simulink model "CLVF"  (R2020a)
settings: Solver=FixedStepAuto  StartTime=0.0  StopTime=tsim  FixedStep=baseRate  RelTol=1e-3  EnableMultiTasking=on
values from neighbouring files (symbols this model uses):
  a = sqrt(sum(aTimesOVec.^2))    [Run_Initializer.m]    (also in a_max_CLVF2D.m = params(4))
  a_max = 0.4/BLACKMass    [Run_Initializer.m]
  a_prime = newParams(2)    [Run_Initializer.m]    (also in a_max_LVF.m = params(2))
  acceptableRadius = 0.05    [Run_Initializer.m]
  b = newParams(3)    [Run_Initializer.m]    (also in a_max_CLVF2D.m = params(3))
  baseRate = 0.05    [Run_Initializer.m]
  BLACKMass = model_param(3)    [Run_Initializer.m]
  d = [0.16;0.542;0]    [Run_Initializer.m]    (also in a_max_LVF.m = [rotStuff(3);rotStuff(4);rotStuff(5)])
  drop_states_BLACK = rC_I0    [Run_Initializer.m]
  drop_states_BLUE = [ xLength/2+0.9; yLength/2+0.5; 0]    [Run_Initializer.m]
  drop_states_RED = rT_I0    [Run_Initializer.m]
  F_thrusters_BLACK = 0.25.*ones(8,1)    [Run_Initializer.m]
  F_thrusters_BLUE = 0.25.*ones(8,1)    [Run_Initializer.m]
  F_thrusters_RED = 0.25.*ones(8,1)    [Run_Initializer.m]
  home_states_BLACK = [ xLength/2+0.4; yLength/2; 0]    [Run_Initializer.m]
  home_states_BLUE = [ xLength/2-0.9; yLength/2+0.5; 0]    [Run_Initializer.m]
  home_states_RED = [ xLength/2-0.4; yLength/2; 0]    [Run_Initializer.m]
  init_states_BLACK = rC_I0    [Run_Initializer.m]
  init_states_BLUE = [ xLength/2+0.9; yLength/2+0.5; 0]    [Run_Initializer.m]
  init_states_RED = rT_I0    [Run_Initializer.m]
  k_v_rel = 2*v_max/a_prime    (= 1)    [Run_Initializer.m]
  ka = newParams(2)    [Run_Initializer.m]    (also in a_max_CLVF2D.m = params(2))
  kc = newParams(1)    [Run_Initializer.m]    (also in a_max_CLVF2D.m = params(1))
  kd = 5.0    (= 5)    [Run_Initializer.m]
  Kd_tb = 0.4    [Run_Initializer.m]
  Kd_tblue = 0.4    [Run_Initializer.m]
  Kd_tr = 0.4    [Run_Initializer.m]
  Kd_xb = 5    [Run_Initializer.m]
  Kd_xblue = 5    [Run_Initializer.m]
  Kd_xr = 5    [Run_Initializer.m]
  Kd_yb = 5    [Run_Initializer.m]
  Kd_yblue = 5    [Run_Initializer.m]
  Kd_yr = 5    [Run_Initializer.m]
  Kp_tb = 0.1    [Run_Initializer.m]
  Kp_tblue = 0.1    [Run_Initializer.m]
  Kp_tr = 0.1    [Run_Initializer.m]
  Kp_xb = 2    [Run_Initializer.m]
  Kp_xblue = 2    [Run_Initializer.m]
  Kp_xr = 2    [Run_Initializer.m]
  Kp_yb = 2    [Run_Initializer.m]
  Kp_yblue = 2    [Run_Initializer.m]
  Kp_yr = 2    [Run_Initializer.m]
  noise_variance_BLACK = 0    [Run_Initializer.m]
  noise_variance_BLUE = 0    [Run_Initializer.m]
  noise_variance_RED = 0    [Run_Initializer.m]
  o_hat_B = aTimesOVec./a    [Run_Initializer.m]
  o_hat_prime = o_prime/sqrt(sum(o_prime.^2))    [Run_Initializer.m]
  Phase0_End = Phase0_Duration    (= 10)    [Run_Initializer.m]
  Phase1_End = Phase0_Duration + Phase1_Duration    (= 15)    [Run_Initializer.m]
  Phase2_End = Phase0_Duration + Phase1_Duration +                                   Phase2_Duration    (= 35)    [Run_Initializer.m]
  Phase3_End = Phase0_Duration + Phase1_Duration +                                   Phase2_Duration + Phase3_Duration    [Run_Initializer.m]
  Phase3_SubPhase1_End = Phase2_End + Phase3_SubPhase1_Duration    (= 40)    [Run_Initializer.m]
  Phase3_SubPhase2_End = Phase2_End + Phase3_SubPhase1_Duration +                                   Phase3_SubPhase2_Duration    (= 45)    [Run_Initializer.m]
  Phase3_SubPhase3_End_BLACK = Phase2_End + Phase3_SubPhase1_Duration +                                   Phase3_SubPhase2_Duration +                                  Phase3_SubPhase3_Duration + Phase3_SubPhase3_and_a_half    (= 51)    [Run_Initializer.m]
  Phase3_SubPhase3_End_RED = Phase2_End + Phase3_SubPhase1_Duration +                                   Phase3_SubPhase2_Duration +                                  Phase3_SubPhase3_Duration    (= 46)    [Run_Initializer.m]
  Phase3_SubPhase4_End = Phase2_End + Phase3_SubPhase1_Duration +                                   Phase3_SubPhase2_Duration +                                  Phase3_SubPhase3_Duration +                                  Phase3_SubPhase4_Duration + Phase3_SubPhase3_and_a_half    [Run_Initializer.m]
  Phase4_End = Phase0_Duration + Phase1_Duration +                                   Phase2_Duration + Phase3_Duration +                                   Phase4_Duration    [Run_Initializer.m]
  Phase5_End = Phase0_Duration + Phase1_Duration +                                   Phase2_Duration + Phase3_Duration +                                   Phase4_Duration + Phase5_Duration    [Run_Initializer.m]
  r_co = r_co_over_a_prime*a_prime    (= 0.16)    [Run_Initializer.m]
  rC_I0 = [0.9*xLength;yLength/2-0.5;pi/2]    [Run_Initializer.m]
  rT_I0 = [yLength/2;yLength/2;possibleStarts(startingRotation)]    [Run_Initializer.m]
  serverRate = 0.1    [Run_Initializer.m]
  sys_BLACK = c2d(sys_BLACK_CONT, baseRate)    [Run_Initializer.m]
  sys_BLACK_ROT = c2d(sys_BLACK_rot_CONT, baseRate)    [Run_Initializer.m]
  sys_RED = c2d(sys_RED_CONT, baseRate)    [Run_Initializer.m]
  sys_RED_ROT = c2d(sys_RED_rot_CONT, baseRate)    [Run_Initializer.m]
  theta_d = 30*d2r    (= 0.523598775598)    [Run_Initializer.m]    (also in a_max_LVF.m = rotStuff(2))
  thruster_dist2CG_BLACK = [83.42;-52.58;55.94;-60.05;54.08;-53.92;77.06;-55.94]    [Run_Initializer.m]
  thruster_dist2CG_BLUE = [83.42;-52.58;55.94;-60.05;54.08;-53.92;77.06;-55.94]    [Run_Initializer.m]
  thruster_dist2CG_RED = [49.92;-78.08;70.46;-63.54;81.08;-50.42;57.44;-75.96]    [Run_Initializer.m]
  w_body = 6.0 * d2r    (= 0.10471975512)    [Run_Initializer.m]
undefined symbols (not defined in the file or in its folder): DiscIntNeverNeededParam, Discrete, Phase3_SubPhase3_End, platformSelection, simMode, Time, WhoAmI
libraries: dspstat3 x18, dspsigops x14, raspberrypiBasiclib x10, embdlinuxlib x8, simulink x8, ctrlSharedLib x4, mspfiltlib x3, dsparch4 x3, dspswit3 x2, MainLibrary x2, sensehatlib x1
(part 2 of 10)

== system CLVF/Phase #3: Experiment ==
  note: In this subsection, the "if" statements are used to determine two things: 1) whether or not a simulation is begin performed,
      | then 2) if an experiment is being performed, then which platform is the diagram compiled on. The "IdentifyPlatform" variable
      | is obtained from a text file location on each platform; each text file contains a unique identifier for each platform.
  Action Port : ActionPort  ActionPortLabel=elseif( u1 < u5)
  Change BLACK Behavior : Subsystem  TreatAsAtomicUnit=on
  Change BLUE Behavior : Subsystem  TreatAsAtomicUnit=on
  Change RED Behavior : Subsystem  TreatAsAtomicUnit=on
  Constant : Constant  Value=WhoAmI
  Is this a simulation? : Subsystem
  This IF block determines whether or not to run the BLACK sim/exp : If  NumInputs=2  IfExpression=u1 == 2 | u2 == 1  ShowElse=off
  This IF block determines whether or not to run the BLUE sim/exp : If  NumInputs=2  IfExpression=u1 == 3 | u2 == 1  ShowElse=off
  "This IF block determines whether or not to run the RED sim/exp " : If  NumInputs=2  IfExpression=u1 == 1 | u2 == 1  ShowElse=off
  wires:
  "This IF block determines whether or not to run the RED sim/exp "/1 -> Change RED Behavior/Action
  This IF block determines whether or not to run the BLACK sim/exp/1 -> Change BLACK Behavior/Action
  Constant/1 -> This IF block determines whether or not to run the BLUE sim/exp/1, This IF block determines whether or not to run the BLACK sim/exp/1, "This IF block determines whether or not to run the RED sim/exp "/1
  Is this a simulation?/1(isSim) -> This IF block determines whether or not to run the BLUE sim/exp/2, This IF block determines whether or not to run the BLACK sim/exp/2, "This IF block determines whether or not to run the RED sim/exp "/2
  This IF block determines whether or not to run the BLUE sim/exp/1 -> Change BLUE Behavior/Action

== system CLVF/Phase #4: Return Home ==
  note: In this subsection, the "if" statements are used to determine two things: 1) whether or not a simulation is begin performed,
      | then 2) if an experiment is being performed, then which platform is the diagram compiled on. The "IdentifyPlatform" variable
      | is obtained from a text file location on each platform; each text file contains a unique identifier for each platform.
  Action Port : ActionPort  ActionPortLabel=elseif( u1 < u6)
  Change BLACK Behavior : Subsystem  TreatAsAtomicUnit=on
  Change BLUE Behavior : Subsystem  TreatAsAtomicUnit=on
  Change RED Behavior : Subsystem  TreatAsAtomicUnit=on
  Constant : Constant  Value=WhoAmI
  Is this a simulation? : Subsystem
  This IF block determines whether or not to run the BLACK sim/exp : If  NumInputs=2  IfExpression=u1 == 2 | u2 == 1  ShowElse=off
  This IF block determines whether or not to run the BLUE sim/exp : If  NumInputs=2  IfExpression=u1 == 3 | u2 == 1  ShowElse=off
  "This IF block determines whether or not to run the RED sim/exp " : If  NumInputs=2  IfExpression=u1 == 1 | u2 == 1  ShowElse=off
  wires:
  "This IF block determines whether or not to run the RED sim/exp "/1 -> Change RED Behavior/Action
  This IF block determines whether or not to run the BLACK sim/exp/1 -> Change BLACK Behavior/Action
  Constant/1 -> This IF block determines whether or not to run the BLUE sim/exp/1, This IF block determines whether or not to run the BLACK sim/exp/1, "This IF block determines whether or not to run the RED sim/exp "/1
  Is this a simulation?/1(isSim) -> This IF block determines whether or not to run the BLUE sim/exp/2, This IF block determines whether or not to run the BLACK sim/exp/2, "This IF block determines whether or not to run the RED sim/exp "/2
  This IF block determines whether or not to run the BLUE sim/exp/1 -> Change BLUE Behavior/Action

== system CLVF/Phase #5: Hold Home ==
  note: In this subsection, the "if" statements are used to determine two things: 1) whether or not a simulation is begin performed,
      | then 2) if an experiment is being performed, then which platform is the diagram compiled on. The "IdentifyPlatform" variable
      | is obtained from a text file location on each platform; each text file contains a unique identifier for each platform.
  note: To change the behavior of RED during this phase, double click on the "Change RED Behavior". For BLACK, double click on "Change BLACK Behavior"
  Action Port : ActionPort  ActionPortLabel=elseif( u1 < u7 )
  Change BLACK Behavior : Subsystem  TreatAsAtomicUnit=on
  Change BLUE Behavior : Subsystem  TreatAsAtomicUnit=on
  Change RED Behavior : Subsystem  TreatAsAtomicUnit=on
  Constant : Constant  Value=WhoAmI
  Is this a simulation? : Subsystem
  This IF block determines whether or not to run the BLACK sim/exp : If  NumInputs=2  IfExpression=u1 == 2 | u2 == 1  ShowElse=off
  This IF block determines whether or not to run the BLUE sim/exp : If  NumInputs=2  IfExpression=u1 == 3 | u2 == 1  ShowElse=off
  "This IF block determines whether or not to run the RED sim/exp " : If  NumInputs=2  IfExpression=u1 == 1 | u2 == 1  ShowElse=off
  wires:
  "This IF block determines whether or not to run the RED sim/exp "/1 -> Change RED Behavior/Action
  This IF block determines whether or not to run the BLACK sim/exp/1 -> Change BLACK Behavior/Action
  Constant/1 -> This IF block determines whether or not to run the BLUE sim/exp/1, This IF block determines whether or not to run the BLACK sim/exp/1, "This IF block determines whether or not to run the RED sim/exp "/1
  This IF block determines whether or not to run the BLUE sim/exp/1 -> Change BLUE Behavior/Action
  Is this a simulation?/1(isSim) -> This IF block determines whether or not to run the BLACK sim/exp/2, This IF block determines whether or not to run the BLUE sim/exp/2, "This IF block determines whether or not to run the RED sim/exp "/2

== system CLVF/Phase #6: Stop Floating and Spin Down RW ==
  note: In this subsection, the "if" statements are used to determine two things: 1) whether or not a simulation is begin performed,
      | then 2) if an experiment is being performed, then which platform is the diagram compiled on. The "IdentifyPlatform" variable
      | is obtained from a text file location on each platform; each text file contains a unique identifier for each platform.
  Action Port : ActionPort  ActionPortLabel=else
  Change BLACK Behavior : Subsystem  TreatAsAtomicUnit=on
  Change BLUE Behavior : Subsystem  TreatAsAtomicUnit=on
  Change RED Behavior : Subsystem  TreatAsAtomicUnit=on
  Constant : Constant  Value=WhoAmI
  Is this a simulation? : Subsystem
  This IF block determines whether or not to run the BLACK sim/exp : If  NumInputs=2  IfExpression=u1 == 2 | u2 == 1  ShowElse=off
  This IF block determines whether or not to run the BLUE sim/exp : If  NumInputs=2  IfExpression=u1 == 3 | u2 == 1  ShowElse=off
  "This IF block determines whether or not to run the RED sim/exp " : If  NumInputs=2  IfExpression=u1 == 1 | u2 == 1  ShowElse=off
  wires:
  "This IF block determines whether or not to run the RED sim/exp "/1 -> Change RED Behavior/Action
  This IF block determines whether or not to run the BLACK sim/exp/1 -> Change BLACK Behavior/Action
  Is this a simulation?/1(isSim) -> This IF block determines whether or not to run the BLUE sim/exp/2, This IF block determines whether or not to run the BLACK sim/exp/2, "This IF block determines whether or not to run the RED sim/exp "/2
  This IF block determines whether or not to run the BLUE sim/exp/1 -> Change BLUE Behavior/Action
  Constant/1 -> This IF block determines whether or not to run the BLACK sim/exp/1, This IF block determines whether or not to run the BLUE sim/exp/1, "This IF block determines whether or not to run the RED sim/exp "/1

== system CLVF/Real-Time Visualization ==
  Set Universal Time (If this is a simulation) : Clock
  UDP Send : embdlinuxlib/UDP Send  remoteURL='192.168.0.105'  remotePort=26000  localURL='0.0.0.0'  localPortSource=Automatically determine  localPort=-1  sampletime=-1  blockPlatform=Raspberry Pi  separateLengthPort=0
      settings: SourceProductBaseCode=SC_BEAGLEBONE_BLUE,RASPPI
  wires:
  Set Universal Time (If this is a simulation)/1 -> UDP Send/1

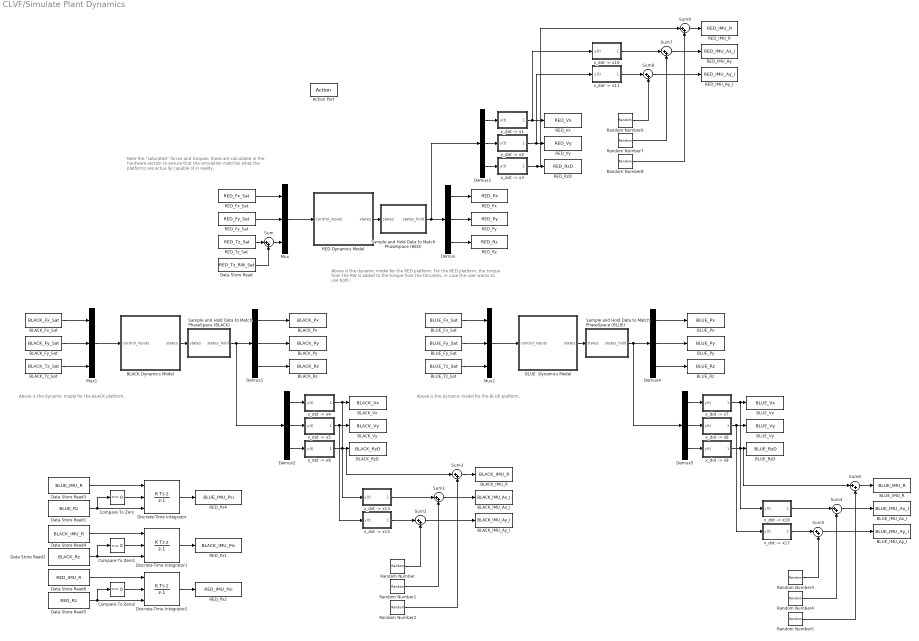
== system CLVF/Simulate Plant Dynamics ==
  note: Above is the dynamic model for the RED
      | platform. For the RED platform, the torque from the RW is added to the torque from the thrusters, in case the user wants to use both.
  note: Above is the dynamic model for the BLACK platform.
  note: Note the "saturated" forces and torques; these are calculated in the hardware section to ensure that the simulation matches what the platforms are actua lly capable of in reality.
  note: Above is the dynamic model for the BLUE platform.
  Action Port : ActionPort  ActionPortLabel=if(u1 == 1)
  BLACK Dynamics Model : Subsystem  SystemSampleTime=serverRate
  BLACK_Fx_Sat : DataStoreRead  DataStoreName=BLACK_Fx_Sat
  BLACK_Fy_Sat : DataStoreRead  DataStoreName=BLACK_Fy_Sat
  BLACK_IMU_Ax_I : DataStoreWrite  DataStoreName=BLACK_IMU_Ax_I
  BLACK_IMU_Ay_I : DataStoreWrite  DataStoreName=BLACK_IMU_Ay_I
  BLACK_IMU_R : DataStoreWrite  DataStoreName=BLACK_IMU_R
  BLACK_Px : DataStoreWrite  DataStoreName=BLACK_Px
  BLACK_Py : DataStoreWrite  DataStoreName=BLACK_Py
  BLACK_Rz : DataStoreWrite  DataStoreName=BLACK_Rz
  BLACK_RzD : DataStoreWrite  DataStoreName=BLACK_RzD
  BLACK_Tz_Sat : DataStoreRead  DataStoreName=BLACK_Tz_Sat
  BLACK_Vx : DataStoreWrite  DataStoreName=BLACK_Vx
  BLACK_Vy : DataStoreWrite  DataStoreName=BLACK_Vy
  BLUE  Dynamics Model : Subsystem  SystemSampleTime=serverRate
  "BLUE_Fx_Sat " : DataStoreRead  DataStoreName=BLUE_Fx_Sat
  BLUE_Fy_Sat : DataStoreRead  DataStoreName=BLUE_Fy_Sat
  BLUE_IMU_Ax_I : DataStoreWrite  DataStoreName=BLUE_IMU_Ax_I
  BLUE_IMU_Ay_I : DataStoreWrite  DataStoreName=BLUE_IMU_Ay_I
  BLUE_IMU_R : DataStoreWrite  DataStoreName=BLUE_IMU_R
  "BLUE_Px " : DataStoreWrite  DataStoreName=BLUE_Px
  BLUE_Py : DataStoreWrite  DataStoreName=BLUE_Py
  BLUE_Rz : DataStoreWrite  DataStoreName=BLUE_Rz
  BLUE_RzD : DataStoreWrite  DataStoreName=BLUE_RzD
  BLUE_Tz_Sat : DataStoreRead  DataStoreName=BLUE_Tz_Sat
  BLUE_Vx : DataStoreWrite  DataStoreName=BLUE_Vx
  BLUE_Vy : DataStoreWrite  DataStoreName=BLUE_Vy
  Compare To Zero : simulink/Logic and Bit Operations/Compare To Zero  relop===  OutDataTypeStr=boolean
  Compare To Zero1 : simulink/Logic and Bit Operations/Compare To Zero  relop===  OutDataTypeStr=boolean
  Compare To Zero2 : simulink/Logic and Bit Operations/Compare To Zero  relop===  OutDataTypeStr=boolean
  Data Store Read : DataStoreRead  DataStoreName=RED_Tz_RW_Sat
  Data Store Read1 : DataStoreRead  DataStoreName=BLUE_Rz
  Data Store Read2 : DataStoreRead  DataStoreName=BLACK_Rz
  Data Store Read3 : DataStoreRead  DataStoreName=BLUE_IMU_R
  Data Store Read4 : DataStoreRead  DataStoreName=BLACK_IMU_R
  Data Store Read5 : DataStoreRead  DataStoreName=RED_Rz
  Data Store Read6 : DataStoreRead  DataStoreName=RED_IMU_R
  Demux{,1..5} (6 alike) : Demux  Outputs=3
  Discrete-Time Integrator : DiscreteIntegrator  IntegratorMethod=Integration: Backward Euler  ExternalReset=either  InitialConditionSource=external  SampleTime=-1  ICPrevOutput=DiscIntNeverNeededParam  ICPrevScaledInput=DiscIntNeverNeededParam
  Discrete-Time Integrator1 : DiscreteIntegrator  IntegratorMethod=Integration: Backward Euler  ExternalReset=either  InitialConditionSource=external  SampleTime=-1  ICPrevOutput=DiscIntNeverNeededParam  ICPrevScaledInput=DiscIntNeverNeededParam
  Discrete-Time Integrator2 : DiscreteIntegrator  IntegratorMethod=Integration: Backward Euler  ExternalReset=either  InitialConditionSource=external  SampleTime=-1  ICPrevOutput=DiscIntNeverNeededParam  ICPrevScaledInput=DiscIntNeverNeededParam
  Mux : Mux  Inputs=3
  Mux1 : Mux  Inputs=3
  Mux2 : Mux  Inputs=3
  RED Dynamics Model : Subsystem  SystemSampleTime=serverRate
  RED_Fx_Sat : DataStoreRead  DataStoreName=RED_Fx_Sat
  RED_Fy_Sat : DataStoreRead  DataStoreName=RED_Fy_Sat
  RED_IMU_Ay : DataStoreWrite  DataStoreName=RED_IMU_Ax_I
  RED_IMU_Ay_I : DataStoreWrite  DataStoreName=RED_IMU_Ay_I
  RED_IMU_R : DataStoreWrite  DataStoreName=RED_IMU_R
  RED_Px : DataStoreWrite  DataStoreName=RED_Px
  RED_Px1 : DataStoreWrite  DataStoreName=BLACK_IMU_Psi
  RED_Px2 : DataStoreWrite  DataStoreName=RED_IMU_Psi
  RED_Px4 : DataStoreWrite  DataStoreName=BLUE_IMU_Psi
  RED_Py : DataStoreWrite  DataStoreName=RED_Py
  RED_Rz : DataStoreWrite  DataStoreName=RED_Rz
  RED_RzD : DataStoreWrite  DataStoreName=RED_RzD
  RED_Tz_Sat : DataStoreRead  DataStoreName=RED_Tz_Sat
  RED_Vx : DataStoreWrite  DataStoreName=RED_Vx
  RED_Vy : DataStoreWrite  DataStoreName=RED_Vy
  Random Number{,1..8} (9 alike) : RandomNumber  Variance=1.5e-6
  Sample and Hold Data to Match PhaseSpace (BLACK) : Subsystem
  Sample and Hold Data to Match PhaseSpace (BLUE) : Subsystem
  Sample and Hold Data to Match PhaseSpace (RED) : Subsystem
  Sum{,1..9} (10 alike) : Sum  Inputs=|++
  "x_dot -> x1" : Subsystem
  "x_dot -> x10" : Subsystem
  "x_dot -> x11" : Subsystem
  "x_dot -> x13" : Subsystem
  "x_dot -> x14" : Subsystem
  "x_dot -> x16" : Subsystem
  "x_dot -> x17" : Subsystem
  "x_dot -> x2" : Subsystem
  "x_dot -> x3" : Subsystem
  "x_dot -> x4" : Subsystem
  "x_dot -> x5" : Subsystem
  "x_dot -> x6" : Subsystem
  "x_dot -> x7" : Subsystem
  "x_dot -> x8" : Subsystem
  "x_dot -> x9" : Subsystem
  wires:
  RED_Fx_Sat/1 -> Mux/1
  BLACK_Fy_Sat/1 -> Mux1/2
  BLACK_Tz_Sat/1 -> Mux1/3
  RED_Fy_Sat/1 -> Mux/2
  BLACK_Fx_Sat/1 -> Mux1/1
  Demux/2 -> RED_Py/1
  Demux/1 -> RED_Px/1
  Demux1/1 -> BLACK_Px/1
  Demux1/2 -> BLACK_Py/1
  RED_Tz_Sat/1 -> Sum/1
  Sum/1 -> Mux/3
  Data Store Read/1 -> Sum/2
  Demux2/1 -> "x_dot -> x4"/1(y(t))
  Demux2/2 -> "x_dot -> x5"/1(y(t))
  Demux2/3 -> "x_dot -> x6"/1(y(t))
  Demux3/2 -> "x_dot -> x2"/1(y(t))
  Demux3/1 -> "x_dot -> x1"/1(y(t))
  Demux3/3 -> "x_dot -> x3"/1(y(t))
  "x_dot -> x1"/1(dy(t)/dt) -> "x_dot -> x10"/1(y(t)), RED_Vx/1
  "x_dot -> x2"/1(dy(t)/dt) -> "x_dot -> x11"/1(y(t)), RED_Vy/1
  "x_dot -> x4"/1(dy(t)/dt) -> "x_dot -> x13"/1(y(t)), BLACK_Vx/1
  "x_dot -> x5"/1(dy(t)/dt) -> "x_dot -> x14"/1(y(t)), BLACK_Vy/1
  "x_dot -> x6"/1(dy(t)/dt) -> Sum3/1, BLACK_RzD/1
  Mux/1 -> RED Dynamics Model/1(control_inputs)
  Mux1/1 -> BLACK Dynamics Model/1(control_inputs)
  Sample and Hold Data to Match PhaseSpace (BLACK)/1(states_hold) -> Demux2/1, Demux1/1
  BLACK Dynamics Model/1(states) -> Sample and Hold Data to Match PhaseSpace (BLACK)/1(states)
  Sample and Hold Data to Match PhaseSpace (RED)/1("states_hold ") -> Demux3/1, Demux/1
  RED Dynamics Model/1(states) -> Sample and Hold Data to Match PhaseSpace (RED)/1(states)
  Demux4/3 -> BLUE_Rz/1
  Demux5/3 -> "x_dot -> x9"/1(y(t))
  Demux4/1 -> "BLUE_Px "/1
  BLUE  Dynamics Model/1(states) -> Sample and Hold Data to Match PhaseSpace (BLUE)/1(states)
  Sample and Hold Data to Match PhaseSpace (BLUE)/1(states_hold) -> Demux5/1, Demux4/1
  "BLUE_Fx_Sat "/1 -> Mux2/1
  BLUE_Fy_Sat/1 -> Mux2/2
  BLUE_Tz_Sat/1 -> Mux2/3
  Mux2/1 -> BLUE  Dynamics Model/1(control_inputs)
  Demux5/1 -> "x_dot -> x7"/1(y(t))
  Demux5/2 -> "x_dot -> x8"/1(y(t))
  Demux4/2 -> BLUE_Py/1
  Demux/3 -> RED_Rz/1
  "x_dot -> x8"/1(dy(t)/dt) -> BLUE_Vy/1, "x_dot -> x17"/1(y(t))
  "x_dot -> x7"/1(dy(t)/dt) -> "x_dot -> x16"/1(y(t)), BLUE_Vx/1
  Demux1/3 -> BLACK_Rz/1
  Discrete-Time Integrator1/1 -> RED_Px1/1
  Discrete-Time Integrator/1 -> RED_Px4/1
  Data Store Read1/1 -> Compare To Zero/1, Discrete-Time Integrator/3
  Compare To Zero/1 -> Discrete-Time Integrator/2
  Data Store Read3/1 -> Discrete-Time Integrator/1
  Data Store Read6/1 -> Discrete-Time Integrator2/1
  Discrete-Time Integrator2/1 -> RED_Px2/1
  Compare To Zero2/1 -> Discrete-Time Integrator2/2
  Data Store Read4/1 -> Discrete-Time Integrator1/1
  Compare To Zero1/1 -> Discrete-Time Integrator1/2
  Data Store Read2/1 -> Compare To Zero1/1, Discrete-Time Integrator1/3
  Data Store Read5/1 -> Compare To Zero2/1, Discrete-Time Integrator2/3
  Sum1/1 -> BLACK_IMU_Ax_I/1
  "x_dot -> x13"/1(dy(t)/dt) -> Sum1/1
  Sum2/1 -> BLACK_IMU_Ay_I/1
  Sum3/1 -> BLACK_IMU_R/1
  Random Number/1 -> Sum2/2
  Random Number1/1 -> Sum1/2
  Random Number2/1 -> Sum3/2
  "x_dot -> x14"/1(dy(t)/dt) -> Sum2/1
  Sum4/1 -> BLUE_IMU_Ax_I/1
  Sum5/1 -> BLUE_IMU_Ay_I/1
  Sum6/1 -> BLUE_IMU_R/1
  "x_dot -> x17"/1(dy(t)/dt) -> Sum5/1
  Random Number3/1 -> Sum5/2
  "x_dot -> x9"/1(dy(t)/dt) -> Sum6/1, BLUE_RzD/1
  "x_dot -> x16"/1(dy(t)/dt) -> Sum4/1
  Random Number5/1 -> Sum6/2
  Random Number4/1 -> Sum4/2
  Sum7/1 -> RED_IMU_Ay/1
  Sum8/1 -> RED_IMU_Ay_I/1
  Sum9/1 -> RED_IMU_R/1
  "x_dot -> x11"/1(dy(t)/dt) -> Sum8/1
  Random Number6/1 -> Sum8/2
  "x_dot -> x3"/1(dy(t)/dt) -> Sum9/1, RED_RzD/1
  "x_dot -> x10"/1(dy(t)/dt) -> Sum7/1
  Random Number8/1 -> Sum9/2
  Random Number7/1 -> Sum7/2

== system CLVF/Subsystem ==
  Universal_Time : DataStoreRead  DataStoreName=Univ_Time
  Time : Outport  VectorParamsAs1DForOutWhenUnconnected=off
  wires:
  Universal_Time/1 -> Time/1

== system CLVF/Float & Magnet Controls/Change Behavior ==
  Action Port : ActionPort  ActionPortLabel=if(u1 == 0)
  Data Store Read : DataStoreRead  DataStoreName=Magnet_State
  Data Store Read1 : DataStoreRead  DataStoreName=Float_State
  GPIO for Magnet : embdlinuxlib/GPIO Write  board=Pi 3 Model B  gpio=10  direction=Output  blockPlatform=Raspberry Pi
      settings: SourceProductBaseCode=SC_BEAGLEBONE_BLUE,RASPPI
  GPIO for Pucks : embdlinuxlib/GPIO Write  board=Pi 3 Model B  gpio=26  direction=Output  blockPlatform=Raspberry Pi
      settings: SourceProductBaseCode=SC_BEAGLEBONE_BLUE,RASPPI
  wires:
  Data Store Read1/1 -> GPIO for Pucks/1
  Data Store Read/1 -> GPIO for Magnet/1

== system CLVF/Float & Magnet Controls/Is this a simulation? ==
  Constant : Constant  Value=simMode  SampleTime=-1
  isSim : Outport  VectorParamsAs1DForOutWhenUnconnected=off
  wires:
  Constant/1 -> isSim/1

== system CLVF/From Force//Torque to PWM Signal/Change BLACK Behavior ==
  note: Calculate the percentage of time each thruster must be on, and send to the PWM blocks.
  note: Using the attitude, rotate the forces into the body frame.
  note: Calculate which thrusters must be turned on and for how long.
  Action Port : ActionPort  ActionPortLabel=if(u1 == 2 | u2 == 1)
  BLACK_Fx : DataStoreRead  DataStoreName=BLACK_Fx
  BLACK_Fy : DataStoreRead  DataStoreName=BLACK_Fy
  BLACK_Rz : DataStoreRead  DataStoreName=BLACK_Rz
  BLACK_Tz : DataStoreRead  DataStoreName=BLACK_Tz
  Calculate Thruster ON/OFF : Subsystem
  Mux : Mux  Inputs=2
  Mux1 : Mux  Inputs=2
  Rotate Forces to Body : Subsystem
  BLACK PWM : Outport  VectorParamsAs1DForOutWhenUnconnected=off
  wires:
  Rotate Forces to Body/1(F_b) -> Mux1/1
  BLACK_Fx/1 -> Mux/1
  Calculate Thruster ON/OFF/1(ThrusterPWM) -> BLACK PWM/1
  BLACK_Rz/1 -> Rotate Forces to Body/2(Rz)
  Mux/1 -> Rotate Forces to Body/1("F_I ")
  BLACK_Tz/1 -> Mux1/2
  Mux1/1 -> Calculate Thruster ON/OFF/1("[Fx_b; Fy_b; Tz]")
  BLACK_Fy/1 -> Mux/2

== system CLVF/From Force//Torque to PWM Signal/Change BLUE Behavior ==
  note: Calculate the percentage of time each thruster must be on, and send to the PWM blocks.
  note: Using the attitude, rotate the forces into the body frame.
  note: Calculate which thrusters must be turned on and for how long.
  Action Port : ActionPort  ActionPortLabel=if(u1 == 3 | u2 == 1)
  BLUE_Fx : DataStoreRead  DataStoreName=BLUE_Fx
  BLUE_Fy : DataStoreRead  DataStoreName=BLUE_Fy
  BLUE_Rz : DataStoreRead  DataStoreName=BLUE_Rz
  BLUE_Tz : DataStoreRead  DataStoreName=BLUE_Tz
  Calculate Thruster ON/OFF : Subsystem
  Mux : Mux  Inputs=2
  Mux1 : Mux  Inputs=2
  Rotate Forces to Body : Subsystem
  BLUE PWM : Outport  VectorParamsAs1DForOutWhenUnconnected=off
  wires:
  Rotate Forces to Body/1(F_b) -> Mux1/1
  BLUE_Fx/1 -> Mux/1
  Calculate Thruster ON/OFF/1(ThrusterPWM) -> BLUE PWM/1
  BLUE_Rz/1 -> Rotate Forces to Body/2(Rz)
  Mux/1 -> Rotate Forces to Body/1("F_I ")
  BLUE_Tz/1 -> Mux1/2
  Mux1/1 -> Calculate Thruster ON/OFF/1("[Fx_b; Fy_b; Tz]")
  BLUE_Fy/1 -> Mux/2

== system CLVF/From Force//Torque to PWM Signal/Change RED Behavior ==
  note: Calculate which thrusters must be turned on and for how long.
  note: Using the attitude, rotate the forces into the body frame.
  note: Calculate the percentage of time each thruster must be on, and send to the PWM blocks.
  Action Port : ActionPort  ActionPortLabel=if(u1 == 1 | u2 == 1)
  Calculate Thruster ON/OFF : Subsystem
  Mux : Mux  Inputs=2
  Mux1 : Mux  Inputs=2
  RED_Fx : DataStoreRead  DataStoreName=RED_Fx
  RED_Fy : DataStoreRead  DataStoreName=RED_Fy
  RED_Rz : DataStoreRead  DataStoreName=RED_Rz
  RED_Tz : DataStoreRead  DataStoreName=RED_Tz
  Rotate Forces to Body : Subsystem
  RED PWM : Outport  VectorParamsAs1DForOutWhenUnconnected=off
  wires:
  RED_Tz/1 -> Mux1/2
  Mux/1 -> Rotate Forces to Body/1("F_I ")
  RED_Fy/1 -> Mux/2
  Mux1/1 -> Calculate Thruster ON/OFF/1("[Fx_b; Fy_b; Tz]")
  RED_Fx/1 -> Mux/1
  RED_Rz/1 -> Rotate Forces to Body/2(Rz)
  Rotate Forces to Body/1(F_b) -> Mux1/1
  Calculate Thruster ON/OFF/1(ThrusterPWM) -> RED PWM/1

== system CLVF/From Force//Torque to PWM Signal/Is this a simulation? ==
  Constant : Constant  Value=simMode  SampleTime=-1
  isSim : Outport  VectorParamsAs1DForOutWhenUnconnected=off
  wires:
  Constant/1 -> isSim/1

== system CLVF/From Force//Torque to PWM Signal/Send Commands to PWM Blocks ==
  In1 : Inport
  In2 : Inport  Port=2
  In3 : Inport  Port=3
  In4 : Inport  Port=4
  In5 : Inport  Port=5
  In6 : Inport  Port=6
  In7 : Inport  Port=7
  In8 : Inport  Port=8
  In9 : Inport  Port=9
  BLACK T2 : raspberrypiBasiclib/PWM  board=Pi 3 Model B  Pin_=9  Frequency=10  blockPlatform=Raspberry Pi
      settings: SourceProductBaseCode=RASPPI
  RED T1 - BLACK T8 : raspberrypiBasiclib/PWM  board=Pi 3 Model B  Pin_=27  Frequency=10  blockPlatform=Raspberry Pi
      settings: SourceProductBaseCode=RASPPI
  RED T2 - BLACK T3 : raspberrypiBasiclib/PWM  board=Pi 3 Model B  Pin_=19  Frequency=10  blockPlatform=Raspberry Pi
      settings: SourceProductBaseCode=RASPPI
  RED T3 : raspberrypiBasiclib/PWM  board=Pi 3 Model B  Pin_=4  Frequency=10  blockPlatform=Raspberry Pi
      settings: SourceProductBaseCode=RASPPI
  RED T4 - BLACK T5 : raspberrypiBasiclib/PWM  board=Pi 3 Model B  Pin_=22  Frequency=10  blockPlatform=Raspberry Pi
      settings: SourceProductBaseCode=RASPPI
  RED T5 - BLACK T4 : raspberrypiBasiclib/PWM  board=Pi 3 Model B  Pin_=5  Frequency=10  blockPlatform=Raspberry Pi
      settings: SourceProductBaseCode=RASPPI
  RED T6 - BLACK T7 : raspberrypiBasiclib/PWM  board=Pi 3 Model B  Pin_=6  Frequency=10  blockPlatform=Raspberry Pi
      settings: SourceProductBaseCode=RASPPI
  RED T7 - BLACK T6 : raspberrypiBasiclib/PWM  board=Pi 3 Model B  Pin_=13  Frequency=10  blockPlatform=Raspberry Pi
      settings: SourceProductBaseCode=RASPPI
  RED T8 - BLACK T1 : raspberrypiBasiclib/PWM  board=Pi 3 Model B  Pin_=17  Frequency=10  blockPlatform=Raspberry Pi
      settings: SourceProductBaseCode=RASPPI
  wires:
  In4/1 -> RED T4 - BLACK T5/1
  In5/1 -> RED T5 - BLACK T4/1
  In1/1 -> RED T1 - BLACK T8/1
  In8/1 -> RED T8 - BLACK T1/1
  In9/1 -> BLACK T2/1
  In7/1 -> RED T7 - BLACK T6/1
  In6/1 -> RED T6 - BLACK T7/1
  In3/1 -> RED T3/1
  In2/1 -> RED T2 - BLACK T3/1

== system CLVF/From Torque, Command RW/Change BLACK Behavior ==
  note: BLACK does not currently have the capability to use a RW.
  Action Port : ActionPort  ActionPortLabel=if(u1 == 2 | u2 == 1)

== system CLVF/From Torque, Command RW/Change BLUE Behavior ==
  note: BLUE does not currently have the capability to use a RW.
  Action Port : ActionPort  ActionPortLabel=if(u1 == 3 | u2 == 1)

== system CLVF/From Torque, Command RW/Change RED Behavior ==
  note: In this subsection, the commanded torque is converted to an RPM, which is then saturated based on the known limits of the RW
  note: The saturated wheel RPM is then sent to the wheel controller using PWM blocks.
  Action Port : ActionPort  ActionPortLabel=if(u1 == 1 | u2 == 1)
  Calculate Saturated RPM Signal : Subsystem
  RED_Tz_RW : DataStoreRead  DataStoreName=RED_Tz_RW
  RED_Tz_RW_Sat : DataStoreWrite  DataStoreName=RED_Tz_RW_Sat
  Wheel RPM to PWM : Subsystem
  wires:
  Calculate Saturated RPM Signal/2(RPM_Sat) -> RED_Tz_RW_Sat/1
  RED_Tz_RW/1 -> Calculate Saturated RPM Signal/1(Tz)
  Calculate Saturated RPM Signal/1(RPM) -> Wheel RPM to PWM/1(WheelRPM)

== system CLVF/From Torque, Command RW/Is this a simulation? ==
  Constant : Constant  Value=simMode  SampleTime=-1
  isSim : Outport  VectorParamsAs1DForOutWhenUnconnected=off
  wires:
  Constant/1 -> isSim/1

== system CLVF/Grab PhaseSpace Data via UDP/Initialize Universal Time (Simulation) ==
  Action Port : ActionPort
  Set Universal Time (If this is a simulation) : Clock
  Universal_Time : DataStoreWrite  DataStoreName=Univ_Time
  wires:
  Set Universal Time (If this is a simulation)/1 -> Universal_Time/1

== system CLVF/Grab PhaseSpace Data via UDP/Is this a simulation?1 ==
  Constant : Constant  Value=simMode  SampleTime=-1
  isSim : Outport  VectorParamsAs1DForOutWhenUnconnected=off
  wires:
  Constant/1 -> isSim/1

== system CLVF/Grab PhaseSpace Data via UDP/Use Hardware to Obtain States ==
  note: Because the UDP block binds to the first platofrm that it sees, it is not currently possible to run RED+BLACK without having RED send BLACK the data packets.
  Action Port : ActionPort
  "Check whether both platforms are being used, and if so then use RED to send data to BLACK " : If  IfExpression=u1 == 1 | u1 == 2 | u1 == 5  ElseIfExpressions=u1 == 3| u1 == 4  ShowElse=off
  "Using RED+BLACK, or RED+BLACK+ARM" : Subsystem  TreatAsAtomicUnit=on
  "Using RED, BLACK, BLUE, or RED + ARM" : Subsystem  TreatAsAtomicUnit=on
  Which PLATFORM is being used? : Constant  Value=platformSelection  SampleTime=-1
  wires:
  "Check whether both platforms are being used, and if so then use RED to send data to BLACK "/1 -> "Using RED, BLACK, BLUE, or RED + ARM"/Action
  "Check whether both platforms are being used, and if so then use RED to send data to BLACK "/2 -> "Using RED+BLACK, or RED+BLACK+ARM"/Action
  Which PLATFORM is being used?/1 -> "Check whether both platforms are being used, and if so then use RED to send data to BLACK "/1

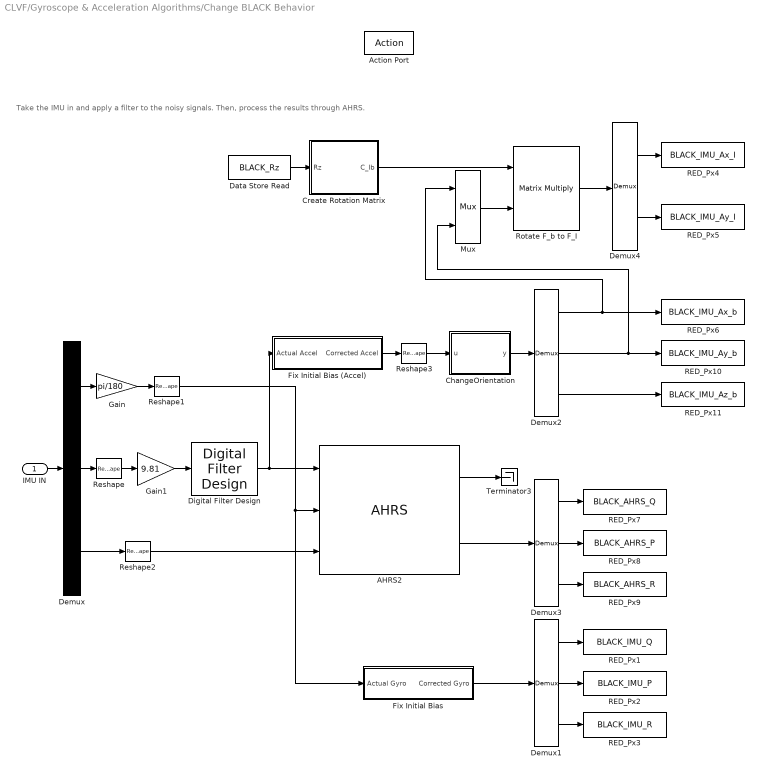
== system CLVF/Gyroscope & Acceleration Algorithms/Change BLACK Behavior ==
  note: Take the IMU in and apply a filter to the noisy signals. Then, process the results through AHRS.
  IMU IN : Inport
  Action Port : ActionPort
  AHRS2 : mspfiltlib/AHRS  DispRefFrame=NED  DecimationFactor=1  InitialProcessNoise=ahrsfilter.defaultProcessNoise  OrientationFormat=quaternion  SimulateUsing=Interpreted execution  AccelerometerNoise=0.0001924722  GyroscopeNoise=9.1385e-5  MagnetometerNoise=0.1  GyroscopeDriftNoise=3.0462e-13  LinearAccelerationNoise=0.0096236100000000012  MagneticDisturbanceNoise=0.5  LinearAccelerationDecayFactor=0.5  MagneticDisturbanceDecayFactor=0.5  ExpectedMagneticFieldStrength=33
      settings: SourceProductBaseCode=TF,NV
  ChangeOrientation : MATLAB Function  TreatAsAtomicUnit=on
  Create Rotation Matrix : MATLAB Function  TreatAsAtomicUnit=on
  Data Store Read : DataStoreRead  DataStoreName=BLACK_Rz
  Demux : Demux  Outputs=[3,3,3]
  Demux1 : Demux  Outputs=3
  Demux2 : Demux  Outputs=3
  Demux3 : Demux  Outputs=3
  Demux4 : Demux  Outputs=2
  Digital Filter Design : dsparch4/Digital Filter Design  mwdsp_browser_bugfix_var=off
  Fix Initial Bias : Subsystem
  Fix Initial Bias (Accel) : Subsystem
  Gain : Gain  Gain=pi/180
  Gain1 : Gain  Gain=9.81
  Mux : Mux  Inputs=2
  RED_Px1 : DataStoreWrite  DataStoreName=BLACK_IMU_Q
  RED_Px10 : DataStoreWrite  DataStoreName=BLACK_IMU_Ay_b
  RED_Px11 : DataStoreWrite  DataStoreName=BLACK_IMU_Az_b
  RED_Px2 : DataStoreWrite  DataStoreName=BLACK_IMU_P
  RED_Px3 : DataStoreWrite  DataStoreName=BLACK_IMU_R
  RED_Px4 : DataStoreWrite  DataStoreName=BLACK_IMU_Ax_I
  RED_Px5 : DataStoreWrite  DataStoreName=BLACK_IMU_Ay_I
  RED_Px6 : DataStoreWrite  DataStoreName=BLACK_IMU_Ax_b
  RED_Px7 : DataStoreWrite  DataStoreName=BLACK_AHRS_Q
  RED_Px8 : DataStoreWrite  DataStoreName=BLACK_AHRS_P
  RED_Px9 : DataStoreWrite  DataStoreName=BLACK_AHRS_R
  Reshape{,1..3} (4 alike) : Reshape  OutputDimensionality=Row vector (2-D)
  Rotate F_b to F_I : Product  Multiplication=Matrix(*)
  Terminator3 : Terminator
  wires:
  Demux3/2 -> RED_Px8/1
  Reshape/1 -> Gain1/1
  Demux3/1 -> RED_Px7/1
  AHRS2/1 -> Terminator3/1
  AHRS2/2 -> Demux3/1
  Demux3/3 -> RED_Px9/1
  Gain/1 -> Reshape1/1
  Demux2/3 -> RED_Px11/1
  Reshape2/1 -> AHRS2/3
  Demux/1 -> Gain/1
  Demux/2 -> Reshape/1
  IMU IN/1 -> Demux/1
  Demux/3 -> Reshape2/1
  Demux1/2 -> RED_Px2/1
  Fix Initial Bias/1(Corrected Gyro) -> Demux1/1
  Demux1/1 -> RED_Px1/1
  Fix Initial Bias (Accel)/1(Corrected Accel) -> Reshape3/1
  Demux1/3 -> RED_Px3/1
  ChangeOrientation/1(y) -> Demux2/1
  Gain1/1 -> Digital Filter Design/1
  Reshape3/1 -> ChangeOrientation/1(u)
  Digital Filter Design/1 -> Fix Initial Bias (Accel)/1(Actual Accel), AHRS2/1
  Reshape1/1 -> Fix Initial Bias/1(Actual Gyro), AHRS2/2
  Create Rotation Matrix/1(C_Ib) -> Rotate F_b to F_I/1
  Rotate F_b to F_I/1 -> Demux4/1
  Mux/1 -> Rotate F_b to F_I/2
  Data Store Read/1 -> Create Rotation Matrix/1(Rz)
  Demux4/1 -> RED_Px4/1
  Demux2/2 -> Mux/2, RED_Px10/1
  Demux2/1 -> Mux/1, RED_Px6/1
  Demux4/2 -> RED_Px5/1

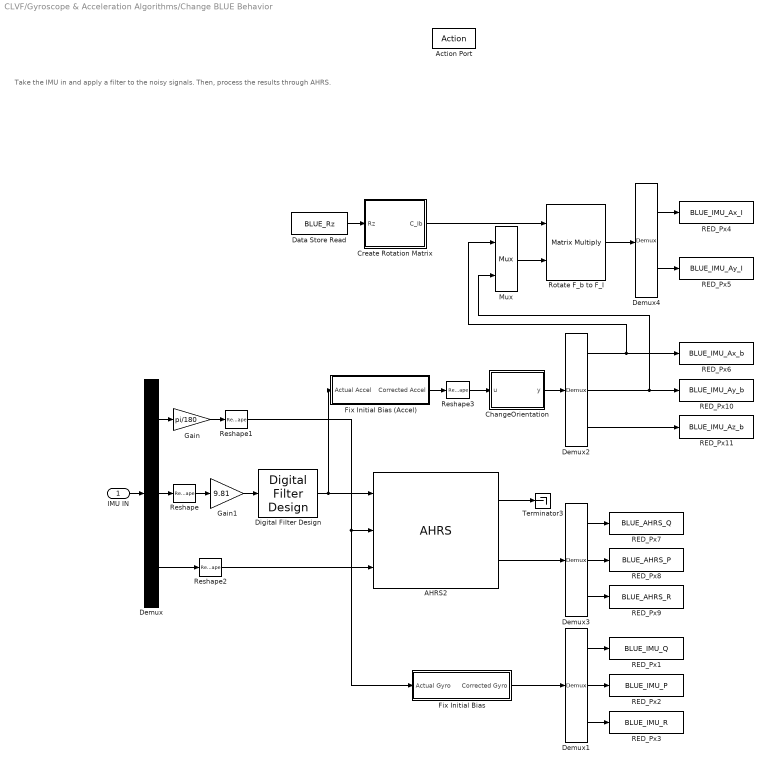
== system CLVF/Gyroscope & Acceleration Algorithms/Change BLUE Behavior ==
  note: Take the IMU in and apply a filter to the noisy signals. Then, process the results through AHRS.
  IMU IN : Inport
  Action Port : ActionPort
  AHRS2 : mspfiltlib/AHRS  DispRefFrame=NED  DecimationFactor=1  InitialProcessNoise=ahrsfilter.defaultProcessNoise  OrientationFormat=quaternion  SimulateUsing=Interpreted execution  AccelerometerNoise=0.0001924722  GyroscopeNoise=9.1385e-5  MagnetometerNoise=0.1  GyroscopeDriftNoise=3.0462e-13  LinearAccelerationNoise=0.0096236100000000012  MagneticDisturbanceNoise=0.5  LinearAccelerationDecayFactor=0.5  MagneticDisturbanceDecayFactor=0.5  ExpectedMagneticFieldStrength=33
      settings: SourceProductBaseCode=TF,NV
  ChangeOrientation : MATLAB Function  TreatAsAtomicUnit=on
  Create Rotation Matrix : MATLAB Function  TreatAsAtomicUnit=on
  Data Store Read : DataStoreRead  DataStoreName=BLUE_Rz
  Demux : Demux  Outputs=[3,3,3]
  Demux1 : Demux  Outputs=3
  Demux2 : Demux  Outputs=3
  Demux3 : Demux  Outputs=3
  Demux4 : Demux  Outputs=2
  Digital Filter Design : dsparch4/Digital Filter Design  mwdsp_browser_bugfix_var=off
  Fix Initial Bias : Subsystem
  Fix Initial Bias (Accel) : Subsystem
  Gain : Gain  Gain=pi/180
  Gain1 : Gain  Gain=9.81
  Mux : Mux  Inputs=2
  RED_Px1 : DataStoreWrite  DataStoreName=BLUE_IMU_Q
  RED_Px10 : DataStoreWrite  DataStoreName=BLUE_IMU_Ay_b
  RED_Px11 : DataStoreWrite  DataStoreName=BLUE_IMU_Az_b
  RED_Px2 : DataStoreWrite  DataStoreName=BLUE_IMU_P
  RED_Px3 : DataStoreWrite  DataStoreName=BLUE_IMU_R
  RED_Px4 : DataStoreWrite  DataStoreName=BLUE_IMU_Ax_I
  RED_Px5 : DataStoreWrite  DataStoreName=BLUE_IMU_Ay_I
  RED_Px6 : DataStoreWrite  DataStoreName=BLUE_IMU_Ax_b
  RED_Px7 : DataStoreWrite  DataStoreName=BLUE_AHRS_Q
  RED_Px8 : DataStoreWrite  DataStoreName=BLUE_AHRS_P
  RED_Px9 : DataStoreWrite  DataStoreName=BLUE_AHRS_R
  Reshape{,1..3} (4 alike) : Reshape  OutputDimensionality=Row vector (2-D)
  Rotate F_b to F_I : Product  Multiplication=Matrix(*)
  Terminator3 : Terminator
  wires:
  Demux/2 -> Reshape/1
  Demux1/1 -> RED_Px1/1
  Gain1/1 -> Digital Filter Design/1
  Fix Initial Bias (Accel)/1(Corrected Accel) -> Reshape3/1
  Demux1/3 -> RED_Px3/1
  Reshape/1 -> Gain1/1
  Fix Initial Bias/1(Corrected Gyro) -> Demux1/1
  Reshape3/1 -> ChangeOrientation/1(u)
  Demux1/2 -> RED_Px2/1
  Demux/3 -> Reshape2/1
  IMU IN/1 -> Demux/1
  Reshape2/1 -> AHRS2/3
  Gain/1 -> Reshape1/1
  Demux3/2 -> RED_Px8/1
  AHRS2/1 -> Terminator3/1
  Demux3/1 -> RED_Px7/1
  Digital Filter Design/1 -> Fix Initial Bias (Accel)/1(Actual Accel), AHRS2/1
  Reshape1/1 -> Fix Initial Bias/1(Actual Gyro), AHRS2/2
  Rotate F_b to F_I/1 -> Demux4/1
  Mux/1 -> Rotate F_b to F_I/2
  Demux4/1 -> RED_Px4/1
  ChangeOrientation/1(y) -> Demux2/1
  Demux/1 -> Gain/1
  Demux2/1 -> Mux/1, RED_Px6/1
  Data Store Read/1 -> Create Rotation Matrix/1(Rz)
  Demux2/2 -> Mux/2, RED_Px10/1
  Demux2/3 -> RED_Px11/1
  Demux4/2 -> RED_Px5/1
  Demux3/3 -> RED_Px9/1
  AHRS2/2 -> Demux3/1
  Create Rotation Matrix/1(C_Ib) -> Rotate F_b to F_I/1

== system CLVF/Gyroscope & Acceleration Algorithms/Change RED Behavior ==
  note: Take the IMU in and apply a filter to the noisy signals. Then, process the results through AHRS.
  IMU IN : Inport
  Action Port : ActionPort
  AHRS2 : mspfiltlib/AHRS  DispRefFrame=NED  DecimationFactor=1  InitialProcessNoise=ahrsfilter.defaultProcessNoise  OrientationFormat=quaternion  SimulateUsing=Interpreted execution  AccelerometerNoise=0.0001924722  GyroscopeNoise=9.1385e-5  MagnetometerNoise=0.1  GyroscopeDriftNoise=3.0462e-13  LinearAccelerationNoise=0.0096236100000000012  MagneticDisturbanceNoise=0.5  LinearAccelerationDecayFactor=0.5  MagneticDisturbanceDecayFactor=0.5  ExpectedMagneticFieldStrength=33
      settings: SourceProductBaseCode=TF,NV
  ChangeOrientation : MATLAB Function  TreatAsAtomicUnit=on
  Create Rotation Matrix : MATLAB Function  TreatAsAtomicUnit=on
  Data Store Read : DataStoreRead  DataStoreName=RED_Rz
  Demux : Demux  Outputs=[3,3,3]
  Demux1 : Demux  Outputs=3
  Demux2 : Demux  Outputs=3
  Demux3 : Demux  Outputs=3
  Demux4 : Demux  Outputs=2
  Digital Filter Design1 : dsparch4/Digital Filter Design  mwdsp_browser_bugfix_var=off
  Fix Initial Bias : Subsystem
  Fix Initial Bias (Accel) : Subsystem
  Gain : Gain  Gain=pi/180
  Gain1 : Gain  Gain=9.81
  Mux : Mux  Inputs=2
  RED_Px1 : DataStoreWrite  DataStoreName=RED_IMU_Q
  RED_Px10 : DataStoreWrite  DataStoreName=RED_IMU_Ax_b
  RED_Px11 : DataStoreWrite  DataStoreName=RED_IMU_Ay_b
  RED_Px12 : DataStoreWrite  DataStoreName=RED_IMU_Az_b
  RED_Px2 : DataStoreWrite  DataStoreName=RED_IMU_P
  RED_Px3 : DataStoreWrite  DataStoreName=RED_IMU_R
  RED_Px4 : DataStoreWrite  DataStoreName=RED_IMU_Ax_I
  RED_Px5 : DataStoreWrite  DataStoreName=RED_IMU_Ay_I
  RED_Px7 : DataStoreWrite  DataStoreName=RED_AHRS_P
  RED_Px8 : DataStoreWrite  DataStoreName=RED_AHRS_Q
  RED_Px9 : DataStoreWrite  DataStoreName=RED_AHRS_R
  Reshape{,1..3} (4 alike) : Reshape  OutputDimensionality=Row vector (2-D)
  Rotate F_b to F_I : Product  Multiplication=Matrix(*)
  Terminator3 : Terminator
  wires:
  Reshape2/1 -> AHRS2/3
  Gain/1 -> Reshape1/1
  Demux2/3 -> RED_Px12/1
  Demux3/3 -> RED_Px9/1
  AHRS2/2 -> Demux3/1
  AHRS2/1 -> Terminator3/1
  Reshape/1 -> Gain1/1
  Demux/2 -> Reshape/1
  Demux/3 -> Reshape2/1
  Demux/1 -> Gain/1
  IMU IN/1 -> Demux/1
  Demux1/1 -> RED_Px1/1
  Demux1/2 -> RED_Px2/1
  Demux1/3 -> RED_Px3/1
  Fix Initial Bias/1(Corrected Gyro) -> Demux1/1
  ChangeOrientation/1(y) -> Demux2/1
  Demux3/2 -> RED_Px7/1
  Demux3/1 -> RED_Px8/1
  Digital Filter Design1/1 -> Fix Initial Bias (Accel)/1(Actual Accel), AHRS2/1
  Gain1/1 -> Digital Filter Design1/1
  Reshape3/1 -> ChangeOrientation/1(u)
  Fix Initial Bias (Accel)/1(Corrected Accel) -> Reshape3/1
  Reshape1/1 -> Fix Initial Bias/1(Actual Gyro), AHRS2/2
  Data Store Read/1 -> Create Rotation Matrix/1(Rz)
  Mux/1 -> Rotate F_b to F_I/2
  Rotate F_b to F_I/1 -> Demux4/1
  Create Rotation Matrix/1(C_Ib) -> Rotate F_b to F_I/1
  Demux2/2 -> Mux/2, RED_Px11/1
  Demux4/1 -> RED_Px4/1
  Demux4/2 -> RED_Px5/1
  Demux2/1 -> Mux/1, RED_Px10/1

== system CLVF/Gyroscope & Acceleration Algorithms/Is this a simulation? ==
  Constant : Constant  Value=simMode  SampleTime=-1
  isSim : Outport  VectorParamsAs1DForOutWhenUnconnected=off
  wires:
  Constant/1 -> isSim/1

== system CLVF/Phase #0: Wait for Synchronization/Change BLACK Behavior ==
  note: Before getting good data, the platforms must NOT be floating. So, float is set to be "off".
  note: For the initialization phase, we do not want any thrust. Thus, all commanded forces are zero.
  Action Port : ActionPort  ActionPortLabel=if(u1 == 2 | u2 == 1)
  BLACK_Fx : DataStoreWrite  DataStoreName=BLACK_Fx
  BLACK_Fy : DataStoreWrite  DataStoreName=BLACK_Fy
  BLACK_Tz : DataStoreWrite  DataStoreName=BLACK_Tz
  Constant3 : Constant  Value=0
  Constant4 : Constant  Value=0
  Constant5 : Constant  Value=0
  Data Store Write4 : DataStoreWrite  DataStoreName=Float_State
  Puck State : Constant  Value=0
  wires:
  Constant3/1 -> BLACK_Fx/1
  Constant5/1 -> BLACK_Tz/1
  Constant4/1 -> BLACK_Fy/1
  Puck State/1 -> Data Store Write4/1

== system CLVF/Phase #0: Wait for Synchronization/Change BLUE Behavior ==
  note: Before getting good data, the platforms must NOT be floating. So, float is set to be "off".
  note: For the initialization phase, we do not want any thrust. Thus, all commanded forces are zero.
  Action Port : ActionPort  ActionPortLabel=if(u1 == 3 | u2 == 1)
  BLUE_Fx : DataStoreWrite  DataStoreName=BLUE_Fx
  BLUE_Fy : DataStoreWrite  DataStoreName=BLUE_Fy
  BLUE_Tz : DataStoreWrite  DataStoreName=BLUE_Tz
  Constant3 : Constant  Value=0
  Constant4 : Constant  Value=0
  Constant5 : Constant  Value=0
  Data Store Write4 : DataStoreWrite  DataStoreName=Float_State
  Puck State : Constant  Value=0
  wires:
  Constant3/1 -> BLUE_Fx/1
  Constant5/1 -> BLUE_Tz/1
  Constant4/1 -> BLUE_Fy/1
  Puck State/1 -> Data Store Write4/1

== system CLVF/Phase #0: Wait for Synchronization/Change RED Behavior ==
  note: For the initialization phase, we do not want any thrust or movement from the robotic arm. Thus, all commanded forces are zero.
  note: Before getting good data, the platforms must NOT be floating. So, float is set to be "off".
  Action Port : ActionPort  ActionPortLabel=if(u1 == 1 | u2 == 1)
  Constant{,1..6} (7 alike) : Constant  Value=0
  Data Store Write : DataStoreWrite  DataStoreName=RED_Tz_Shoulder
  Data Store Write1 : DataStoreWrite  DataStoreName=RED_Tz_Elbow
  Data Store Write2 : DataStoreWrite  DataStoreName=RED_Tz_Wrist
  Data Store Write4 : DataStoreWrite  DataStoreName=Float_State
  Puck State : Constant  Value=0
  RED_Fx : DataStoreWrite  DataStoreName=RED_Fx
  RED_Fy : DataStoreWrite  DataStoreName=RED_Fy
  RED_Tz : DataStoreWrite  DataStoreName=RED_Tz
  RED_Tz_RW : DataStoreWrite  DataStoreName=RED_Tz_RW
  wires:
  Constant1/1 -> RED_Fy/1
  Constant2/1 -> RED_Tz/1
  Constant/1 -> RED_Fx/1
  Constant4/1 -> Data Store Write/1
  Constant5/1 -> Data Store Write1/1
  Constant6/1 -> Data Store Write2/1
  Constant3/1 -> RED_Tz_RW/1
  Puck State/1 -> Data Store Write4/1

== system CLVF/Phase #0: Wait for Synchronization/Is this a simulation? ==
  Constant : Constant  Value=simMode  SampleTime=-1
  isSim : Outport  VectorParamsAs1DForOutWhenUnconnected=off
  wires:
  Constant/1 -> isSim/1

== system CLVF/Phase #1: Start Floating /Change BLACK Behavior ==
  note: For the float phase, we do not want any thrust. Thus, all commanded forces are zero.
  note: Now that good data is available, the platform can start to float.
  Action Port : ActionPort  ActionPortLabel=if(u1 == 2 | u2 == 1)
  BLACK_Fx : DataStoreWrite  DataStoreName=BLACK_Fx
  BLACK_Fy : DataStoreWrite  DataStoreName=BLACK_Fy
  BLACK_Tz : DataStoreWrite  DataStoreName=BLACK_Tz
  Constant3 : Constant  Value=0
  Constant4 : Constant  Value=0
  Constant5 : Constant  Value=0
  Data Store Write4 : DataStoreWrite  DataStoreName=Float_State
  Puck State : Constant
  wires:
  Constant3/1 -> BLACK_Fx/1
  Constant5/1 -> BLACK_Tz/1
  Constant4/1 -> BLACK_Fy/1
  Puck State/1 -> Data Store Write4/1

== system CLVF/Phase #1: Start Floating /Change BLUE Behavior ==
  note: Before getting good data, the platforms must NOT be floating. So, float is set to be "off".
  note: For the initialization phase, we do not want any thrust. Thus, all commanded forces are zero.
  Action Port : ActionPort  ActionPortLabel=if(u1 == 3 | u2 == 1)
  BLUE_Fx : DataStoreWrite  DataStoreName=BLUE_Fx
  BLUE_Fy : DataStoreWrite  DataStoreName=BLUE_Fy
  BLUE_Tz : DataStoreWrite  DataStoreName=BLUE_Tz
  Constant3 : Constant  Value=0
  Constant4 : Constant  Value=0
  Constant5 : Constant  Value=0
  Data Store Write4 : DataStoreWrite  DataStoreName=Float_State
  Puck State : Constant
  wires:
  Constant3/1 -> BLUE_Fx/1
  Constant5/1 -> BLUE_Tz/1
  Constant4/1 -> BLUE_Fy/1
  Puck State/1 -> Data Store Write4/1

== system CLVF/Phase #1: Start Floating /Change RED Behavior ==
  note: Now that good data is available, the platforms can start to float.
  note: For the float phase, we do not want any thrust or movement from the robotic arm. Thus, all commanded forces are zero.
  Action Port : ActionPort  ActionPortLabel=if(u1 == 1 | u2 == 1)
  Constant{,1..6} (7 alike) : Constant  Value=0
  Data Store Write : DataStoreWrite  DataStoreName=RED_Tz_Shoulder
  Data Store Write1 : DataStoreWrite  DataStoreName=RED_Tz_Elbow
  Data Store Write2 : DataStoreWrite  DataStoreName=RED_Tz_Wrist
  Data Store Write4 : DataStoreWrite  DataStoreName=Float_State
  Puck State : Constant
  RED_Fx : DataStoreWrite  DataStoreName=RED_Fx
  RED_Fy : DataStoreWrite  DataStoreName=RED_Fy
  RED_Tz : DataStoreWrite  DataStoreName=RED_Tz
  RED_Tz_RW : DataStoreWrite  DataStoreName=RED_Tz_RW
  wires:
  Constant/1 -> RED_Fx/1
  Constant3/1 -> RED_Tz_RW/1
  Constant4/1 -> Data Store Write/1
  Constant2/1 -> RED_Tz/1
  Constant6/1 -> Data Store Write2/1
  Constant1/1 -> RED_Fy/1
  Constant5/1 -> Data Store Write1/1
  Puck State/1 -> Data Store Write4/1

== system CLVF/Phase #1: Start Floating /Is this a simulation? ==
  Constant : Constant  Value=simMode  SampleTime=-1
  isSim : Outport  VectorParamsAs1DForOutWhenUnconnected=off
  wires:
  Constant/1 -> isSim/1

== system CLVF/Phase #2: Move to Initial Position/Change BLACK Behavior ==
  note: Additional Blocks
  note: PD Control Law - BLACK
  note: Additional blocks are stored here.
  note: A simple PD control law is used here to command the platform to it's initial position, as defined in the initializer.
  Action Port : ActionPort  ActionPortLabel=if(u1 == 2 | u2 == 1)
  BLACK_Fx : DataStoreWrite  DataStoreName=BLACK_Fx
  BLACK_Fy : DataStoreWrite  DataStoreName=BLACK_Fy
  BLACK_Px : DataStoreRead  DataStoreName=BLACK_Px
  "BLACK_Py " : DataStoreRead  DataStoreName=BLACK_Py
  BLACK_Rz : DataStoreRead  DataStoreName=BLACK_Rz
  BLACK_Tz : DataStoreWrite  DataStoreName=BLACK_Tz
  Custom Discrete PD (Attitude) : Subsystem
  Custom Discrete PD (X-Position) : Subsystem
  Custom Discrete PD (Y-Position) : Subsystem
  Data Store Write3 : DataStoreWrite  DataStoreName=Float_State
  Desired Attitude (BLACK) : Constant  Value=init_states_BLACK(3)  SampleTime=-1
  Desired Px (BLACK) : Constant  Value=init_states_BLACK(1)  SampleTime=-1
  Desired Py (BLACK) : Constant  Value=init_states_BLACK(2)  SampleTime=-1
  Hough Control : Subsystem
  Puck State : Constant
  Subtract : Sum  Inputs=+-
  Subtract1 : Sum  Inputs=+-
  wires:
  Custom Discrete PD (Y-Position)/1(Fy) -> BLACK_Fy/1
  Hough Control/1(Err) -> Custom Discrete PD (Attitude)/1(ez)
  BLACK_Px/1 -> Subtract/2
  Subtract1/1 -> Custom Discrete PD (Y-Position)/1(ey)
  Custom Discrete PD (Attitude)/1(Tz) -> BLACK_Tz/1
  "BLACK_Py "/1 -> Subtract1/2
  Subtract/1 -> Custom Discrete PD (X-Position)/1(ex)
  Custom Discrete PD (X-Position)/1(Fx) -> BLACK_Fx/1
  Desired Px (BLACK)/1 -> Subtract/1
  Desired Py (BLACK)/1 -> Subtract1/1
  Desired Attitude (BLACK)/1 -> Hough Control/1(Ref)
  BLACK_Rz/1 -> Hough Control/2(Act)
  Puck State/1 -> Data Store Write3/1
